simulink model "lr4_v20_task2_d1"  (R2023a)
settings: Solver=FixedStepDiscrete  StartTime=0  StopTime=1  FixedStep=h  RelTol=1e-9  AbsTol=1e-11
InitFcn:
  | h=0.01; a=18; p=2; q=4;
undefined symbols (not defined in the file or in its folder): DiscIntNeverNeededParam
settings Model: Creator=theju  LastModifiedBy=theju

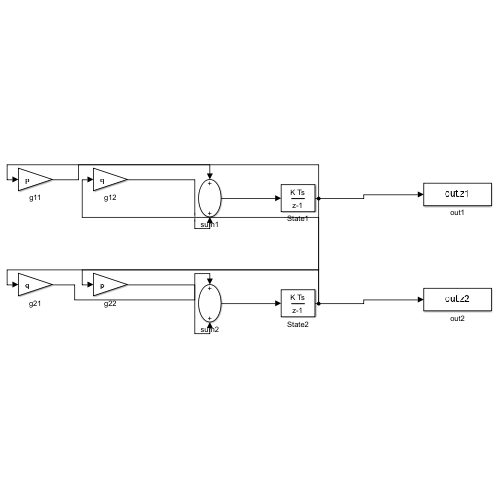
[thumbnail: Simulink's stored preview of the top-level diagram]
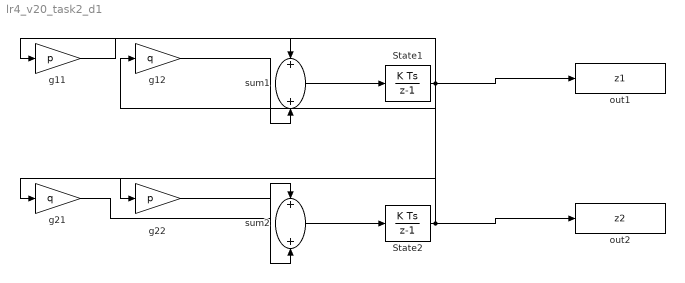
== system lr4_v20_task2_d1 ==
  State1 : DiscreteIntegrator  InitialCondition=3  SampleTime=h  ICPrevOutput=DiscIntNeverNeededParam  ICPrevScaledInput=DiscIntNeverNeededParam
  State2 : DiscreteIntegrator  SampleTime=h  ICPrevOutput=DiscIntNeverNeededParam  ICPrevScaledInput=DiscIntNeverNeededParam
  g11 : Gain  Gain=p
  g12 : Gain  Gain=q
  g21 : Gain  Gain=q
  g22 : Gain  Gain=p
  out1 : ToWorkspace  VariableName=z1  SaveFormat=Timeseries  SampleTime=-1
  out2 : ToWorkspace  VariableName=z2  SaveFormat=Timeseries  SampleTime=-1
  sum1 : Sum
  sum2 : Sum
  wires:
  State1/1 -> out1/1, g11/1, g21/1
  State2/1 -> out2/1, g12/1, g22/1
  g11/1 -> sum1/1
  g12/1 -> sum1/2
  sum1/1 -> State1/1
  g21/1 -> sum2/1
  g22/1 -> sum2/2
  sum2/1 -> State2/1
